simulink model "DAB_RA8P1_Final_Physical_MOSFET"  (R2024b)
settings: Solver=daessc  StartTime=0.0  StopTime=0.03  MaxStep=1e-8  RelTol=2e-3  AbsTol=1e-5
libraries: ee_lib x118, fl_lib x18, nesl_utility x15
(part 1 of 6)
Description:
  | H1.7 physical DAB model. Includes MOS/PCB/TMCS conductor parasitics, TMCS 120 ns + 1.1 MHz measurement path, 250 ns worst-case OC delay, hardware latch abstraction, independent driver enable, and physical-model EPS. TMCS1133B1A hardware mapping: 25 mV/A at 3.3 V; saved OC thresholds 63.728093 A primary and 39.169139 A secondary.
settings Model: Creator=LENOVO  LastModifiedBy=26488

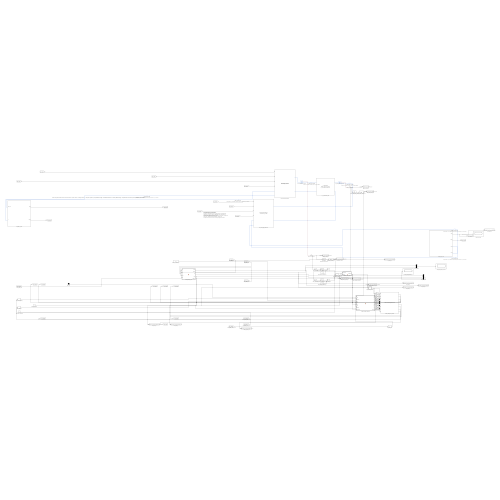
[thumbnail: Simulink's stored preview of the top-level diagram]
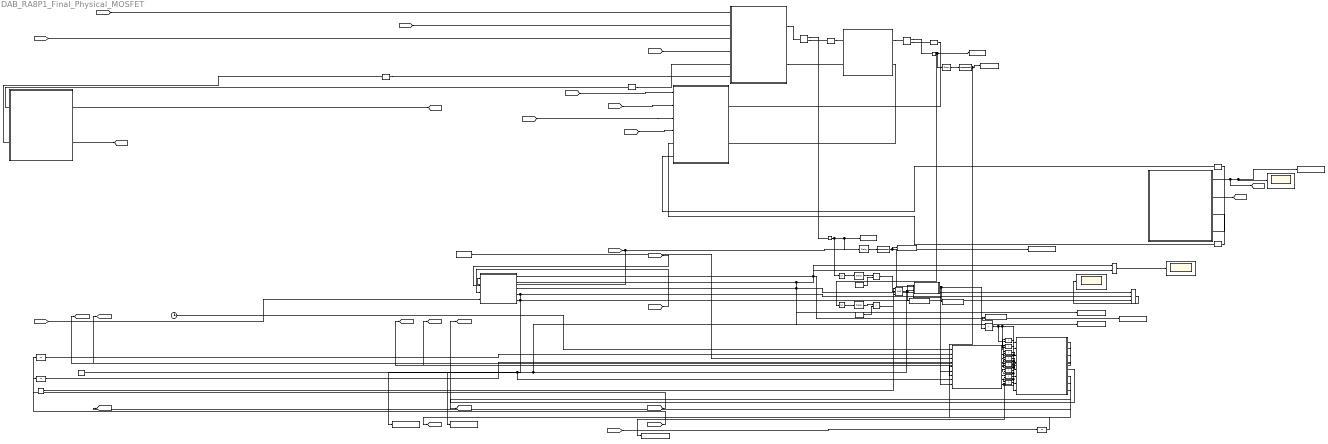
== system DAB_RA8P1_Final_Physical_MOSFET ==
  note: Selected physical parts used in the final model
      | Q1-Q8: AOS AONS66917, 100 V silicon MOSFET.
      | Gate drive: 4x UCC21520DWR, 0/10.18 V, 120 ns MCU dead time, no PNP/NPN booster.
      | Per MOS: Rg_on 4.7 Ohm, Rg_off 2.2 Ohm, PMEG4010ER, Rgs 10 kOhm, BZT52C15.
      | Transformer: custom PQ4040 PC95, Np:Ns=1:2 fixed, L1/L2=57.5/230uH, Llk_sec(total)=0.5uH.
      | Input CM choke only: 2mH per winding, 30A, no bypass.
      | Output: CSEC -> SER2915H-222KL 2.2uH/2.05mOhm -> 8000uF COUT.
      | No output common-mode choke, no common-mode copper bridge, no GaN variant.
  note: Power path: input EMI -> primary MOSFET full bridge -> PQ4040/PC95 transformer -> secondary MOSFET bridge -> output filter/load. Control and scopes are kept below the power schematic.
  note: RA8P1-friendly realtime feedback control: measured Vin/Vout/Iout -> PI phase command -> isolated gate interface.
  ADC_Delay_Iout : UnitDelay  SampleTime=1e-6  HasFrameUpgradeWarning=on
  ADC_Delay_Vin : UnitDelay  InitialCondition=24  SampleTime=1e-6  HasFrameUpgradeWarning=on
  ADC_OneCycle_Delay : UnitDelay  SampleTime=1e-6  HasFrameUpgradeWarning=on
  DRIVER_ENABLE_scope_sl : ToWorkspace  VariableName=DAB_RA8P1_Final_Physical_MOSFET_driver_enable  SaveFormat=Structure With Time  SampleTime=-1
  Eff_scope_sl : ToWorkspace  VariableName=DAB_RA8P1_Final_Physical_MOSFET_efficiency  SaveFormat=Structure With Time  SampleTime=-1
  FAULT_LATCH_N_scope_sl : ToWorkspace  VariableName=DAB_RA8P1_Final_Physical_MOSFET_fault_latch_n  SaveFormat=Structure With Time  SampleTime=-1
  HW_DRIVER_ENABLE : Product
  HW_GATE_Q{1..8} (8 alike) : Product
  Hardware_Fault_Latch_N : MATLAB Function  TreatAsAtomicUnit=on
  IPRI_Abs_For_OC : Abs  SaturateOnIntegerOverflow=off
  IPRI_HF_To_Simulink : nesl_utility/PS-Simulink Converter  PhysicalDomain=network_engine_domain  SubClassName=ps_output  LeftPortType=input  RightPortType=output  PseudoPeriodic=off  Frequencies=[]  VectorFormat=inherit  Unit=inherit  AffineConversion=off
  IPRI_HF_scope_sl : ToWorkspace  VariableName=DAB_RA8P1_Final_Physical_MOSFET_ipri_hf  SaveFormat=Structure With Time
  IPRI_HW_OC_Threshold_A : Constant  Value=63.728093
  IPRI_OC_Safe : RelationalOperator  Operator=<  OutDataTypeStr=boolean  RndMeth=Simplest  InputSameDT=off
  IPRI_TMCS_scope_sl : ToWorkspace  VariableName=DAB_RA8P1_Final_Physical_MOSFET_ipri_tmcs  SaveFormat=Structure With Time  SampleTime=-1
  ISEC_Abs_For_OC : Abs  SaturateOnIntegerOverflow=off
  ISEC_HF_To_Simulink : nesl_utility/PS-Simulink Converter  PhysicalDomain=network_engine_domain  SubClassName=ps_output  LeftPortType=input  RightPortType=output  PseudoPeriodic=off  Frequencies=[]  VectorFormat=inherit  Unit=inherit  AffineConversion=off
  ISEC_HF_scope_sl : ToWorkspace  VariableName=DAB_RA8P1_Final_Physical_MOSFET_isec_hf  SaveFormat=Structure With Time
  ISEC_HW_OC_Threshold_A : Constant  Value=39.169139
  ISEC_OC_Safe : RelationalOperator  Operator=<  OutDataTypeStr=boolean  RndMeth=Simplest  InputSameDT=off
  ISEC_TMCS_scope_sl : ToWorkspace  VariableName=DAB_RA8P1_Final_Physical_MOSFET_isec_tmcs  SaveFormat=Structure With Time  SampleTime=-1
  Iin_scope_sl : ToWorkspace  VariableName=DAB_RA8P1_Final_Physical_MOSFET_iin  SaveFormat=Structure With Time  SampleTime=-1
  Input_EMI_DC_Link : Subsystem
  Iout_scope_sl : ToWorkspace  VariableName=DAB_RA8P1_Final_Physical_MOSFET_iout  SaveFormat=Structure With Time  SampleTime=-1
  Isolated_Gate_Drive_Interface : Subsystem
      mask Display: color('black');disp('UCC21520 isolated gate driver bank');
  LPCB_PRI_NEG_5nH : ee_lib/Passive/Inductor  l=5 nH  enable_L_tol=ee.enum.toleranceApplication.none  L_tol=20  tol_distribution=ee.enum.toleranceDistribution.uniform  nSigma=4  r=0.0001 Ohm  g=1e-9 1/Ohm  enable_operating_limits=ee.enum.enable.no  operating_limit_action=ee.enum.passive.reportOpLim.warn  max_working_current=1 A  power_rating=1 W  fault_action=simscape.enum.assert.action.none  t_fault=1 s  i_L_specify=off  i_L_priority=High  i_L=0 A  i_L_nominal_specify=off  i_L_nominal_value=1  i_L_nominal_unit=A
      settings: AttributesFormatString=PCB parasitic only; not a BOM component; keep PRI local DC loop <=10nH total
  LPCB_PRI_POS_5nH : ee_lib/Passive/Inductor  l=5 nH  enable_L_tol=ee.enum.toleranceApplication.none  L_tol=20  tol_distribution=ee.enum.toleranceDistribution.uniform  nSigma=4  r=0.0001 Ohm  g=1e-9 1/Ohm  enable_operating_limits=ee.enum.enable.no  operating_limit_action=ee.enum.passive.reportOpLim.warn  max_working_current=1 A  power_rating=1 W  fault_action=simscape.enum.assert.action.none  t_fault=1 s  i_L_specify=off  i_L_priority=High  i_L=0 A  i_L_nominal_specify=off  i_L_nominal_value=1  i_L_nominal_unit=A
      settings: AttributesFormatString=PCB parasitic only; not a BOM component; keep PRI local DC loop <=10nH total
  LPCB_SEC_NEG_5nH : ee_lib/Passive/Inductor  l=5 nH  enable_L_tol=ee.enum.toleranceApplication.none  L_tol=20  tol_distribution=ee.enum.toleranceDistribution.uniform  nSigma=4  r=0.0001 Ohm  g=1e-9 1/Ohm  enable_operating_limits=ee.enum.enable.no  operating_limit_action=ee.enum.passive.reportOpLim.warn  max_working_current=1 A  power_rating=1 W  fault_action=simscape.enum.assert.action.none  t_fault=1 s  i_L_specify=off  i_L_priority=High  i_L=0 A  i_L_nominal_specify=off  i_L_nominal_value=1  i_L_nominal_unit=A
      settings: AttributesFormatString=PCB parasitic only; not a BOM component; keep SEC local DC loop <=10nH total
  LPCB_SEC_POS_5nH : ee_lib/Passive/Inductor  l=5 nH  enable_L_tol=ee.enum.toleranceApplication.none  L_tol=20  tol_distribution=ee.enum.toleranceDistribution.uniform  nSigma=4  r=0.0001 Ohm  g=1e-9 1/Ohm  enable_operating_limits=ee.enum.enable.no  operating_limit_action=ee.enum.passive.reportOpLim.warn  max_working_current=1 A  power_rating=1 W  fault_action=simscape.enum.assert.action.none  t_fault=1 s  i_L_specify=off  i_L_priority=High  i_L=0 A  i_L_nominal_specify=off  i_L_nominal_value=1  i_L_nominal_unit=A
      settings: AttributesFormatString=PCB parasitic only; not a BOM component; keep SEC local DC loop <=10nH total
  MCU_Vout_Setpoint_V : Constant  Value=48
  Mux_Currents : Mux  Inputs=2
  Mux_Power_Eff : Mux  Inputs=3
  Output_Filter_Load : Subsystem
  PRI_Full_Bridge_RealDrivers : Subsystem
      mask Display: color('black');disp('PRI Full Bridge RealDrivers\nnonideal FETs + gate RCD');
  Phase_us_scope_sl : ToWorkspace  VariableName=DAB_RA8P1_Final_Physical_MOSFET_phase_us  SaveFormat=Structure With Time  SampleTime=-1
  Pin_scope_sl : ToWorkspace  VariableName=DAB_RA8P1_Final_Physical_MOSFET_pin  SaveFormat=Structure With Time  SampleTime=-1
  Pout_scope_sl : ToWorkspace  VariableName=DAB_RA8P1_Final_Physical_MOSFET_pout  SaveFormat=Structure With Time  SampleTime=-1
  Power_Efficiency_Calc : MATLAB Function  TreatAsAtomicUnit=on
  RA8P1_Realtime_Voltage_PI : MATLAB Function  TreatAsAtomicUnit=on
  RAW_FAULT_N_Model : Constant
  RAW_FAULT_N_With_OC : Logic  Inputs=3  AllPortsSameDT=off  OutDataTypeStr=boolean
  RAW_FAULT_N_scope_sl : ToWorkspace  VariableName=DAB_RA8P1_Final_Physical_MOSFET_raw_fault_n  SaveFormat=Structure With Time  SampleTime=-1
  RUN_REQ_Model : Constant
  R_TMCS_PRI_0p7mOhm : ee_lib/Passive/Resistor  R=0.0007 Ohm  enable_R_tol=ee.enum.toleranceApplication.none  R_tol=5  tol_distribution=ee.enum.toleranceDistribution.uniform  nSigma=4  enable_operating_limits=ee.enum.enable.no  operating_limit_action=ee.enum.passive.reportOpLim.warn  power_rating=1 W  max_working_voltage=100 V  noise_mode=ee.enum.sources.noise.Disabled  Tdevice=25 degC  sample_time=1e-3 s  repeatability=ee.enum.ic.repeatability.notRepeatable  user_seed=0  auto_seed=3499211588  fault_action=simscape.enum.assert.action.none  t_fault=1 s  power_derating_T1=70 degC  power_derating_T2=155 degC  operating_temperature_range_vec=[-50, 150] degC  alpha=3.93e-3 1/K  Tmeas=25 degC  thermal_mass=100 J/K  temperature_specify=off  temperature_priority=High  temperature=298.15 K  temperature_nominal_specify=off  temperature_nominal_value=1  temperature_nominal_unit=K
      settings: AttributesFormatString=TMCS1133 conductor resistance; physical U_IPRI in BOM
  R_TMCS_SEC_0p7mOhm : ee_lib/Passive/Resistor  R=0.0007 Ohm  enable_R_tol=ee.enum.toleranceApplication.none  R_tol=5  tol_distribution=ee.enum.toleranceDistribution.uniform  nSigma=4  enable_operating_limits=ee.enum.enable.no  operating_limit_action=ee.enum.passive.reportOpLim.warn  power_rating=1 W  max_working_voltage=100 V  noise_mode=ee.enum.sources.noise.Disabled  Tdevice=25 degC  sample_time=1e-3 s  repeatability=ee.enum.ic.repeatability.notRepeatable  user_seed=0  auto_seed=3890346746  fault_action=simscape.enum.assert.action.none  t_fault=1 s  power_derating_T1=70 degC  power_derating_T2=155 degC  operating_temperature_range_vec=[-50, 150] degC  alpha=3.93e-3 1/K  Tmeas=25 degC  thermal_mass=100 J/K  temperature_specify=off  temperature_priority=High  temperature=298.15 K  temperature_nominal_specify=off  temperature_nominal_value=1  temperature_nominal_unit=K
      settings: AttributesFormatString=TMCS1133 conductor resistance; physical U_ISEC in BOM
  SEC_Full_Bridge_RealDrivers : Subsystem
      mask Display: color('black');disp('SEC Full Bridge RealDrivers\nnonideal FETs + gate RCD');
  Scope_Input_Output_Current : Scope
  Scope_Power_Efficiency : Scope
  Scope_Vout_Load : Scope
  Sim_Time : Clock
  T1_HF_Transformer_Real : Subsystem
      mask Display: color('black');disp('T1 PQ4040 PC95\nNp:Ns 1:2 fixed, Llk_sec 0.5uH\nLm_sec 230uH, DCR 0.95/3mR');
  TMCS_IPRI_1p1MHz_LPF : TransferFcn  Numerator=[2*pi*1.1e6]  Denominator=[1 2*pi*1.1e6]
  TMCS_IPRI_Analog_Delay : TransportDelay  DelayTime=120e-9
  TMCS_IPRI_OC_WorstCase_Delay : TransportDelay  DelayTime=250e-9
  TMCS_ISEC_1p1MHz_LPF : TransferFcn  Numerator=[2*pi*1.1e6]  Denominator=[1 2*pi*1.1e6]
  TMCS_ISEC_Analog_Delay : TransportDelay  DelayTime=120e-9
  TMCS_ISEC_OC_WorstCase_Delay : TransportDelay  DelayTime=250e-9
  U_IPRI_TMCS1133_Current : fl_lib/Electrical/Electrical Sensors/Current Sensor
  U_ISEC_TMCS1133_Current : fl_lib/Electrical/Electrical Sensors/Current Sensor
  Vin_scope_sl : ToWorkspace  VariableName=DAB_RA8P1_Final_Physical_MOSFET_vin  SaveFormat=Structure With Time  SampleTime=-1
  Vout_scope_sl : ToWorkspace  VariableName=DAB_RA8P1_Final_Physical_MOSFET_vout  SaveFormat=Structure With Time  SampleTime=-1
  wires:
  [VIN_MEAS] -> Power_Efficiency_Calc/1(Vin), Vin_scope_sl/1
  [IIN_MEAS] -> Power_Efficiency_Calc/2(Iin)
  [VOUT_MEAS] -> Power_Efficiency_Calc/3(Vout)
  [IOUT_MEAS] -> Power_Efficiency_Calc/4(Iout)
  Power_Efficiency_Calc/1(IinAbs) -> Iin_scope_sl/1, Mux_Currents/1
  Power_Efficiency_Calc/2(IoutAbs) -> Mux_Currents/2, Iout_scope_sl/1
  Power_Efficiency_Calc/3(Pin) -> Pin_scope_sl/1, Mux_Power_Eff/1
  Power_Efficiency_Calc/4(Pout) -> Pout_scope_sl/1, Mux_Power_Eff/2
  Power_Efficiency_Calc/5(Efficiency) -> Mux_Power_Eff/3, Eff_scope_sl/1
  Mux_Currents/1 -> Scope_Input_Output_Current/1
  Mux_Power_Eff/1 -> Scope_Power_Efficiency/1
  Input_EMI_DC_Link/1(output) -> [IIN_MEAS]
  Input_EMI_DC_Link/2(output1) -> [VIN_MEAS]
  Output_Filter_Load/1(output) -> Vout_scope_sl/1, Scope_Vout_Load/1, [VOUT_MEAS]
  Output_Filter_Load/2(output1) -> [IOUT_MEAS]
  Isolated_Gate_Drive_Interface/1(GATE_OUT_1) -> [Q1_GATE]
  Isolated_Gate_Drive_Interface/2(GATE_OUT_2) -> [Q2_GATE]
  Isolated_Gate_Drive_Interface/3(GATE_OUT_3) -> [Q3_GATE]
  Isolated_Gate_Drive_Interface/4(GATE_OUT_4) -> [Q4_GATE]
  Isolated_Gate_Drive_Interface/5(GATE_OUT_5) -> [Q5_GATE]
  Isolated_Gate_Drive_Interface/6(GATE_OUT_6) -> [Q6_GATE]
  Isolated_Gate_Drive_Interface/7(GATE_OUT_7) -> [Q7_GATE]
  Isolated_Gate_Drive_Interface/8(GATE_OUT_8) -> [Q8_GATE]
  Sim_Time/1 -> RA8P1_Realtime_Voltage_PI/1(t)
  ADC_OneCycle_Delay/1 -> RA8P1_Realtime_Voltage_PI/2(Vout)
  MCU_Vout_Setpoint_V/1 -> RA8P1_Realtime_Voltage_PI/3(VrefCmd)
  [VIN_MEAS] -> ADC_Delay_Vin/1
  ADC_Delay_Vin/1 -> RA8P1_Realtime_Voltage_PI/4(Vin)
  [IOUT_MEAS] -> ADC_Delay_Iout/1
  ADC_Delay_Iout/1 -> RA8P1_Realtime_Voltage_PI/5(Iout)
  RA8P1_Realtime_Voltage_PI/9(PhaseUs) -> Phase_us_scope_sl/1
  [Q1_GATE] -> PRI_Full_Bridge_RealDrivers/1(G1_A_HS)
  [Q2_GATE] -> PRI_Full_Bridge_RealDrivers/2(G2_A_LS)
  [Q3_GATE] -> PRI_Full_Bridge_RealDrivers/3(G3_B_HS)
  [Q4_GATE] -> PRI_Full_Bridge_RealDrivers/4(G4_B_LS)
  [Q5_GATE] -> SEC_Full_Bridge_RealDrivers/1(G1_A_HS)
  [Q6_GATE] -> SEC_Full_Bridge_RealDrivers/2(G2_A_LS)
  [Q7_GATE] -> SEC_Full_Bridge_RealDrivers/3(G3_B_HS)
  [Q8_GATE] -> SEC_Full_Bridge_RealDrivers/4(G4_B_LS)
  [VOUT_MEAS] -> ADC_OneCycle_Delay/1
  RUN_REQ_Model/1 -> Hardware_Fault_Latch_N/2(RunReq), HW_DRIVER_ENABLE/1, RA8P1_Realtime_Voltage_PI/8(RunReq)
  IPRI_HF_To_Simulink/1 -> IPRI_HF_scope_sl/1, TMCS_IPRI_Analog_Delay/1, IPRI_Abs_For_OC/1
  TMCS_IPRI_Analog_Delay/1 -> TMCS_IPRI_1p1MHz_LPF/1
  TMCS_IPRI_1p1MHz_LPF/1 -> RA8P1_Realtime_Voltage_PI/6(Ipri), IPRI_TMCS_scope_sl/1
  ISEC_HF_To_Simulink/1 -> ISEC_HF_scope_sl/1, TMCS_ISEC_Analog_Delay/1, ISEC_Abs_For_OC/1
  TMCS_ISEC_Analog_Delay/1 -> TMCS_ISEC_1p1MHz_LPF/1
  TMCS_ISEC_1p1MHz_LPF/1 -> RA8P1_Realtime_Voltage_PI/7(Isec), ISEC_TMCS_scope_sl/1
  IPRI_Abs_For_OC/1 -> TMCS_IPRI_OC_WorstCase_Delay/1
  TMCS_IPRI_OC_WorstCase_Delay/1 -> IPRI_OC_Safe/1
  IPRI_HW_OC_Threshold_A/1 -> IPRI_OC_Safe/2
  ISEC_Abs_For_OC/1 -> TMCS_ISEC_OC_WorstCase_Delay/1
  TMCS_ISEC_OC_WorstCase_Delay/1 -> ISEC_OC_Safe/1
  ISEC_HW_OC_Threshold_A/1 -> ISEC_OC_Safe/2
  RAW_FAULT_N_Model/1 -> RAW_FAULT_N_With_OC/1
  IPRI_OC_Safe/1 -> RAW_FAULT_N_With_OC/2
  ISEC_OC_Safe/1 -> RAW_FAULT_N_With_OC/3
  RAW_FAULT_N_With_OC/1 -> RAW_FAULT_N_scope_sl/1, Hardware_Fault_Latch_N/1(RawFaultN)
  Hardware_Fault_Latch_N/1(FaultLatchN) -> FAULT_LATCH_N_scope_sl/1, HW_DRIVER_ENABLE/2, RA8P1_Realtime_Voltage_PI/9(RawFaultN)
  HW_DRIVER_ENABLE/1 -> HW_GATE_Q7/2, HW_GATE_Q8/2, HW_GATE_Q6/2, HW_GATE_Q5/2, HW_GATE_Q4/2, HW_GATE_Q3/2, HW_GATE_Q2/2, HW_GATE_Q1/2, DRIVER_ENABLE_scope_sl/1
  RA8P1_Realtime_Voltage_PI/1(g1) -> HW_GATE_Q1/1
  HW_GATE_Q1/1 -> Isolated_Gate_Drive_Interface/1(PWM_IN_1)
  RA8P1_Realtime_Voltage_PI/2(g2) -> HW_GATE_Q2/1
  HW_GATE_Q2/1 -> Isolated_Gate_Drive_Interface/2(PWM_IN_2)
  RA8P1_Realtime_Voltage_PI/3(g3) -> HW_GATE_Q3/1
  HW_GATE_Q3/1 -> Isolated_Gate_Drive_Interface/3(PWM_IN_3)
  RA8P1_Realtime_Voltage_PI/4(g4) -> HW_GATE_Q4/1
  HW_GATE_Q4/1 -> Isolated_Gate_Drive_Interface/4(PWM_IN_4)
  RA8P1_Realtime_Voltage_PI/5(g5) -> HW_GATE_Q5/1
  HW_GATE_Q5/1 -> Isolated_Gate_Drive_Interface/5(PWM_IN_5)
  RA8P1_Realtime_Voltage_PI/6(g6) -> HW_GATE_Q6/1
  HW_GATE_Q6/1 -> Isolated_Gate_Drive_Interface/6(PWM_IN_6)
  RA8P1_Realtime_Voltage_PI/7(g7) -> HW_GATE_Q7/1
  HW_GATE_Q7/1 -> Isolated_Gate_Drive_Interface/7(PWM_IN_7)
  RA8P1_Realtime_Voltage_PI/8(g8) -> HW_GATE_Q8/1
  HW_GATE_Q8/1 -> Isolated_Gate_Drive_Interface/8(PWM_IN_8)
  connections:
  PRI_Full_Bridge_RealDrivers/RConn2 -- T1_HF_Transformer_Real/LConn2
  T1_HF_Transformer_Real/RConn2 -- SEC_Full_Bridge_RealDrivers/RConn2
  Input_EMI_DC_Link/LConn1 -- LPCB_PRI_POS_5nH/LConn1
  LPCB_PRI_POS_5nH/RConn1 -- PRI_Full_Bridge_RealDrivers/LConn1
  Input_EMI_DC_Link/LConn2 -- LPCB_PRI_NEG_5nH/LConn1
  LPCB_PRI_NEG_5nH/RConn1 -- PRI_Full_Bridge_RealDrivers/LConn2
  SEC_Full_Bridge_RealDrivers/LConn1 -- LPCB_SEC_POS_5nH/LConn1
  LPCB_SEC_POS_5nH/RConn1 -- Output_Filter_Load/RConn1
  SEC_Full_Bridge_RealDrivers/LConn2 -- LPCB_SEC_NEG_5nH/LConn1
  LPCB_SEC_NEG_5nH/RConn1 -- Output_Filter_Load/RConn2
  PRI_Full_Bridge_RealDrivers/RConn1 -- U_IPRI_TMCS1133_Current/LConn1
  U_IPRI_TMCS1133_Current/RConn2 -- R_TMCS_PRI_0p7mOhm/LConn1
  R_TMCS_PRI_0p7mOhm/RConn1 -- T1_HF_Transformer_Real/LConn1
  T1_HF_Transformer_Real/RConn1 -- U_ISEC_TMCS1133_Current/LConn1
  U_ISEC_TMCS1133_Current/RConn2 -- R_TMCS_SEC_0p7mOhm/LConn1
  R_TMCS_SEC_0p7mOhm/RConn1 -- SEC_Full_Bridge_RealDrivers/RConn1
  U_IPRI_TMCS1133_Current/RConn1 -- IPRI_HF_To_Simulink/LConn1
  U_ISEC_TMCS1133_Current/RConn1 -- ISEC_HF_To_Simulink/LConn1

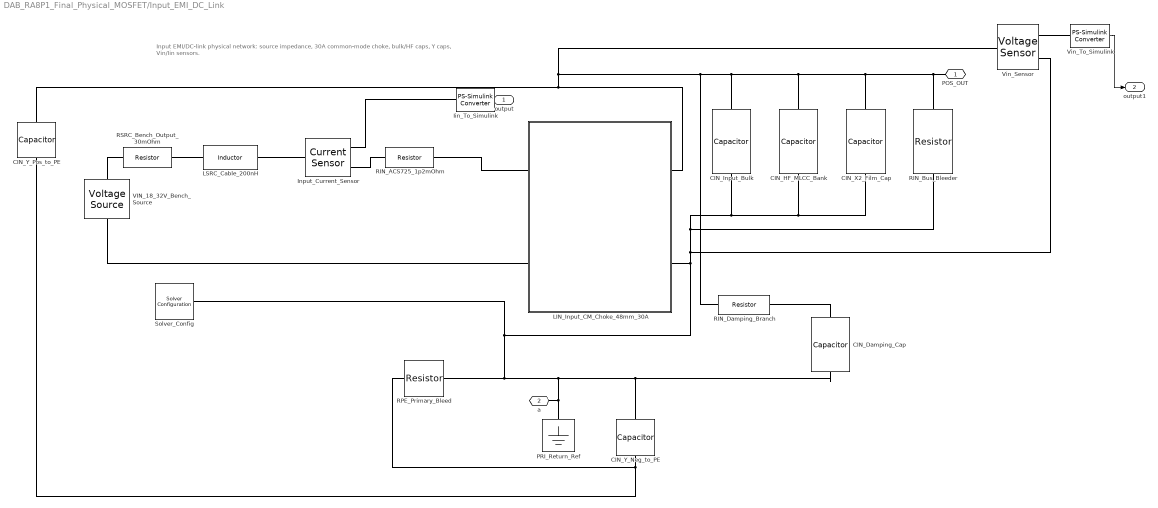
== system DAB_RA8P1_Final_Physical_MOSFET/Input_EMI_DC_Link ==
  note: Input EMI/DC-link physical network: source impedance, 30A common-mode choke, bulk/HF caps, Y caps, Vin/Iin sensors.
  CIN_Damping_Cap : ee_lib/Passive/Capacitor  cap_option=ee.enum.passive.capacitor.capOption.const  c=40 uF  Cvec=[1e-05, 1e-06] F  Vvec=[0, 10] V  CV_table_symmetry=ee.enum.passive.capacitor.tableSymmetry.yes  f_vec=[1, 10] kHz  DFext_vec=[.8, 1.2]  enable_C_tol=ee.enum.toleranceApplication.none  averaging_period=0 s  C_tol=5  tol_distribution=ee.enum.toleranceDistribution.uniform  nSigma=4  r=0.002 Ohm  g=0 1/Ohm  enable_operating_limits=ee.enum.enable.no  operating_limit_action=ee.enum.passive.reportOpLim.warn  max_working_voltage_range=[-25, 25] V  power_rating=1 W  maxTemperature=85 degC  thermalEnable=false  thermalMass=1 J/K  fault_action=simscape.enum.assert.action.none  t_fault=1 s  i_specify=off  i_priority=None  i=0 A  i_nominal_specify=off  i_nominal_value=1  i_nominal_unit=A  v_specify=off  v_priority=None  v=0 V  v_nominal_specify=off  v_nominal_value=1  v_nominal_unit=V  vc_specify=on  vc_priority=High  vc=24 V  vc_nominal_specify=off  vc_nominal_value=1  vc_nominal_unit=V  T_specify=off  T_priority=None  T=298.15 K  T_nominal_specify=off  T_nominal_value=1  T_nominal_unit=K
      settings: AttributesFormatString=110uF
  CIN_HF_MLCC_Bank : ee_lib/Passive/Capacitor  cap_option=ee.enum.passive.capacitor.capOption.const  c=220 uF  Cvec=[1e-05, 1e-06] F  Vvec=[0, 10] V  CV_table_symmetry=ee.enum.passive.capacitor.tableSymmetry.yes  f_vec=[1, 10] kHz  DFext_vec=[.8, 1.2]  enable_C_tol=ee.enum.toleranceApplication.none  averaging_period=0 s  C_tol=5  tol_distribution=ee.enum.toleranceDistribution.uniform  nSigma=4  r=0.0010 Ohm  g=0 1/Ohm  enable_operating_limits=ee.enum.enable.no  operating_limit_action=ee.enum.passive.reportOpLim.warn  max_working_voltage_range=[-25, 25] V  power_rating=1 W  maxTemperature=85 degC  thermalEnable=false  thermalMass=1 J/K  fault_action=simscape.enum.assert.action.none  t_fault=1 s  i_specify=off  i_priority=None  i=0 A  i_nominal_specify=off  i_nominal_value=1  i_nominal_unit=A  v_specify=off  v_priority=None  v=0 V  v_nominal_specify=off  v_nominal_value=1  v_nominal_unit=V  vc_specify=on  vc_priority=High  vc=24 V  vc_nominal_specify=off  vc_nominal_value=1  vc_nominal_unit=V  T_specify=off  T_priority=None  T=298.15 K  T_nominal_specify=off  T_nominal_value=1  T_nominal_unit=K
      settings: AttributesFormatString=220uF\nMLCC
  CIN_Input_Bulk : ee_lib/Passive/Capacitor  cap_option=ee.enum.passive.capacitor.capOption.const  c=4000 uF  Cvec=[1e-05, 1e-06] F  Vvec=[0, 10] V  CV_table_symmetry=ee.enum.passive.capacitor.tableSymmetry.yes  f_vec=[1, 10] kHz  DFext_vec=[.8, 1.2]  enable_C_tol=ee.enum.toleranceApplication.none  averaging_period=0 s  C_tol=5  tol_distribution=ee.enum.toleranceDistribution.uniform  nSigma=4  r=0.006 Ohm  g=0 1/Ohm  enable_operating_limits=ee.enum.enable.no  operating_limit_action=ee.enum.passive.reportOpLim.warn  max_working_voltage_range=[-25, 25] V  power_rating=1 W  maxTemperature=85 degC  thermalEnable=false  thermalMass=1 J/K  fault_action=simscape.enum.assert.action.none  t_fault=1 s  i_specify=off  i_priority=None  i=0 A  i_nominal_specify=off  i_nominal_value=1  i_nominal_unit=A  v_specify=off  v_priority=None  v=0 V  v_nominal_specify=off  v_nominal_value=1  v_nominal_unit=V  vc_specify=on  vc_priority=High  vc=24 V  vc_nominal_specify=off  vc_nominal_value=1  vc_nominal_unit=V  T_specify=off  T_priority=None  T=298.15 K  T_nominal_specify=off  T_nominal_value=1  T_nominal_unit=K
      settings: AttributesFormatString=4000uF\nESR 6mR
  CIN_X2_Film_Cap : ee_lib/Passive/Capacitor  cap_option=ee.enum.passive.capacitor.capOption.const  c=2.2 uF  Cvec=[1e-05, 1e-06] F  Vvec=[0, 10] V  CV_table_symmetry=ee.enum.passive.capacitor.tableSymmetry.yes  f_vec=[1, 10] kHz  DFext_vec=[.8, 1.2]  enable_C_tol=ee.enum.toleranceApplication.none  averaging_period=0 s  C_tol=5  tol_distribution=ee.enum.toleranceDistribution.uniform  nSigma=4  r=0.01 Ohm  g=0 1/Ohm  enable_operating_limits=ee.enum.enable.no  operating_limit_action=ee.enum.passive.reportOpLim.warn  max_working_voltage_range=[-25, 25] V  power_rating=1 W  maxTemperature=85 degC  thermalEnable=false  thermalMass=1 J/K  fault_action=simscape.enum.assert.action.none  t_fault=1 s  i_specify=off  i_priority=None  i=0 A  i_nominal_specify=off  i_nominal_value=1  i_nominal_unit=A  v_specify=off  v_priority=None  v=0 V  v_nominal_specify=off  v_nominal_value=1  v_nominal_unit=V  vc_specify=on  vc_priority=High  vc=24 V  vc_nominal_specify=off  vc_nominal_value=1  vc_nominal_unit=V  T_specify=off  T_priority=None  T=298.15 K  T_nominal_specify=off  T_nominal_value=1  T_nominal_unit=K
      settings: AttributesFormatString=2.2uF film
  CIN_Y_Neg_to_PE : ee_lib/Passive/Capacitor  cap_option=ee.enum.passive.capacitor.capOption.const  c=2.2 nF  Cvec=[1e-05, 1e-06] F  Vvec=[0, 10] V  CV_table_symmetry=ee.enum.passive.capacitor.tableSymmetry.yes  f_vec=[1, 10] kHz  DFext_vec=[.8, 1.2]  enable_C_tol=ee.enum.toleranceApplication.none  averaging_period=0 s  C_tol=5  tol_distribution=ee.enum.toleranceDistribution.uniform  nSigma=4  r=0.02 Ohm  g=0 1/Ohm  enable_operating_limits=ee.enum.enable.no  operating_limit_action=ee.enum.passive.reportOpLim.warn  max_working_voltage_range=[-25, 25] V  power_rating=1 W  maxTemperature=85 degC  thermalEnable=false  thermalMass=1 J/K  fault_action=simscape.enum.assert.action.none  t_fault=1 s  i_specify=off  i_priority=None  i=0 A  i_nominal_specify=off  i_nominal_value=1  i_nominal_unit=A  v_specify=off  v_priority=None  v=0 V  v_nominal_specify=off  v_nominal_value=1  v_nominal_unit=V  vc_specify=off  vc_priority=High  vc=0 V  vc_nominal_specify=off  vc_nominal_value=1  vc_nominal_unit=V  T_specify=off  T_priority=None  T=298.15 K  T_nominal_specify=off  T_nominal_value=1  T_nominal_unit=K
      settings: AttributesFormatString=Y 2.2nF
  CIN_Y_Pos_to_PE : ee_lib/Passive/Capacitor  cap_option=ee.enum.passive.capacitor.capOption.const  c=2.2 nF  Cvec=[1e-05, 1e-06] F  Vvec=[0, 10] V  CV_table_symmetry=ee.enum.passive.capacitor.tableSymmetry.yes  f_vec=[1, 10] kHz  DFext_vec=[.8, 1.2]  enable_C_tol=ee.enum.toleranceApplication.none  averaging_period=0 s  C_tol=5  tol_distribution=ee.enum.toleranceDistribution.uniform  nSigma=4  r=0.02 Ohm  g=0 1/Ohm  enable_operating_limits=ee.enum.enable.no  operating_limit_action=ee.enum.passive.reportOpLim.warn  max_working_voltage_range=[-25, 25] V  power_rating=1 W  maxTemperature=85 degC  thermalEnable=false  thermalMass=1 J/K  fault_action=simscape.enum.assert.action.none  t_fault=1 s  i_specify=off  i_priority=None  i=0 A  i_nominal_specify=off  i_nominal_value=1  i_nominal_unit=A  v_specify=off  v_priority=None  v=0 V  v_nominal_specify=off  v_nominal_value=1  v_nominal_unit=V  vc_specify=off  vc_priority=High  vc=0 V  vc_nominal_specify=off  vc_nominal_value=1  vc_nominal_unit=V  T_specify=off  T_priority=None  T=298.15 K  T_nominal_specify=off  T_nominal_value=1  T_nominal_unit=K
      settings: AttributesFormatString=Y 2.2nF
  Iin_To_Simulink : nesl_utility/PS-Simulink Converter  PhysicalDomain=network_engine_domain  SubClassName=ps_output  LeftPortType=input  RightPortType=output  PseudoPeriodic=off  Frequencies=[]  VectorFormat=inherit  Unit=inherit  AffineConversion=off
  Input_Current_Sensor : fl_lib/Electrical/Electrical Sensors/Current Sensor
      settings: AttributesFormatString=Iin sense
  LIN_Input_CM_Choke_48mm_30A : Subsystem
      mask Display: color('black');disp('48mm CM choke\n2mH, 30A, DCR<=3.5mR\nZcm>2.1k@150kHz');
  LSRC_Cable_200nH : ee_lib/Passive/Inductor  l=0.2 uH  enable_L_tol=ee.enum.toleranceApplication.none  L_tol=20  tol_distribution=ee.enum.toleranceDistribution.uniform  nSigma=4  r=0.003 Ohm  g=1e-9 1/Ohm  enable_operating_limits=ee.enum.enable.no  operating_limit_action=ee.enum.passive.reportOpLim.warn  max_working_current=50 A  power_rating=1 W  fault_action=simscape.enum.assert.action.none  t_fault=1 s  i_L_specify=off  i_L_priority=High  i_L=0 A  i_L_nominal_specify=off  i_L_nominal_value=1  i_L_nominal_unit=A
      settings: AttributesFormatString=200nH\n3mR
  PRI_Return_Ref : fl_lib/Electrical/Electrical Elements/Electrical Reference
  RIN_ACS725_1p2mOhm : ee_lib/Passive/Resistor  R=0.0012 Ohm  enable_R_tol=ee.enum.toleranceApplication.none  R_tol=5  tol_distribution=ee.enum.toleranceDistribution.uniform  nSigma=4  enable_operating_limits=ee.enum.enable.no  operating_limit_action=ee.enum.passive.reportOpLim.warn  power_rating=1 W  max_working_voltage=100 V  noise_mode=ee.enum.sources.noise.Disabled  Tdevice=25 degC  sample_time=1e-3 s  repeatability=ee.enum.ic.repeatability.notRepeatable  user_seed=0  auto_seed=3936355183  fault_action=simscape.enum.assert.action.none  t_fault=1 s  power_derating_T1=70 degC  power_derating_T2=155 degC  operating_temperature_range_vec=[-50, 150] degC  alpha=3.93e-3 1/K  Tmeas=25 degC  thermal_mass=100 J/K  temperature_specify=off  temperature_priority=High  temperature=298.15 K  temperature_nominal_specify=off  temperature_nominal_value=1  temperature_nominal_unit=K
      settings: AttributesFormatString=1mR
  RIN_Bus_Bleeder : ee_lib/Passive/Resistor  R=5000 Ohm  enable_R_tol=ee.enum.toleranceApplication.none  R_tol=5  tol_distribution=ee.enum.toleranceDistribution.uniform  nSigma=4  enable_operating_limits=ee.enum.enable.no  operating_limit_action=ee.enum.passive.reportOpLim.warn  power_rating=1 W  max_working_voltage=100 V  noise_mode=ee.enum.sources.noise.Disabled  Tdevice=25 degC  sample_time=1e-3 s  repeatability=ee.enum.ic.repeatability.notRepeatable  user_seed=0  auto_seed=1207334858  fault_action=simscape.enum.assert.action.none  t_fault=1 s  power_derating_T1=70 degC  power_derating_T2=155 degC  operating_temperature_range_vec=[-50, 150] degC  alpha=3.93e-3 1/K  Tmeas=25 degC  thermal_mass=100 J/K  temperature_specify=off  temperature_priority=High  temperature=298.15 K  temperature_nominal_specify=off  temperature_nominal_value=1  temperature_nominal_unit=K
      settings: AttributesFormatString=100k
  RIN_Damping_Branch : ee_lib/Passive/Resistor  R=0.33 Ohm  enable_R_tol=ee.enum.toleranceApplication.none  R_tol=5  tol_distribution=ee.enum.toleranceDistribution.uniform  nSigma=4  enable_operating_limits=ee.enum.enable.no  operating_limit_action=ee.enum.passive.reportOpLim.warn  power_rating=1 W  max_working_voltage=100 V  noise_mode=ee.enum.sources.noise.Disabled  Tdevice=25 degC  sample_time=1e-3 s  repeatability=ee.enum.ic.repeatability.notRepeatable  user_seed=0  auto_seed=3897705473  fault_action=simscape.enum.assert.action.none  t_fault=1 s  power_derating_T1=70 degC  power_derating_T2=155 degC  operating_temperature_range_vec=[-50, 150] degC  alpha=3.93e-3 1/K  Tmeas=25 degC  thermal_mass=100 J/K  temperature_specify=off  temperature_priority=High  temperature=298.15 K  temperature_nominal_specify=off  temperature_nominal_value=1  temperature_nominal_unit=K
      settings: AttributesFormatString=0.33R
  RPE_Primary_Bleed : ee_lib/Passive/Resistor  R=100000000 Ohm  enable_R_tol=ee.enum.toleranceApplication.none  R_tol=5  tol_distribution=ee.enum.toleranceDistribution.uniform  nSigma=4  enable_operating_limits=ee.enum.enable.no  operating_limit_action=ee.enum.passive.reportOpLim.warn  power_rating=1 W  max_working_voltage=100 V  noise_mode=ee.enum.sources.noise.Disabled  Tdevice=25 degC  sample_time=1e-3 s  repeatability=ee.enum.ic.repeatability.notRepeatable  user_seed=0  auto_seed=477115713  fault_action=simscape.enum.assert.action.none  t_fault=1 s  power_derating_T1=70 degC  power_derating_T2=155 degC  operating_temperature_range_vec=[-50, 150] degC  alpha=3.93e-3 1/K  Tmeas=25 degC  thermal_mass=100 J/K  temperature_specify=off  temperature_priority=High  temperature=298.15 K  temperature_nominal_specify=off  temperature_nominal_value=1  temperature_nominal_unit=K
      settings: AttributesFormatString=100MR
  RSRC_Bench_Output_30mOhm : ee_lib/Passive/Resistor  R=0.03 Ohm  enable_R_tol=ee.enum.toleranceApplication.none  R_tol=5  tol_distribution=ee.enum.toleranceDistribution.uniform  nSigma=4  enable_operating_limits=ee.enum.enable.no  operating_limit_action=ee.enum.passive.reportOpLim.warn  power_rating=1 W  max_working_voltage=100 V  noise_mode=ee.enum.sources.noise.Disabled  Tdevice=25 degC  sample_time=1e-3 s  repeatability=ee.enum.ic.repeatability.notRepeatable  user_seed=0  auto_seed=1331131015  fault_action=simscape.enum.assert.action.none  t_fault=1 s  power_derating_T1=70 degC  power_derating_T2=155 degC  operating_temperature_range_vec=[-50, 150] degC  alpha=3.93e-3 1/K  Tmeas=25 degC  thermal_mass=100 J/K  temperature_specify=off  temperature_priority=High  temperature=298.15 K  temperature_nominal_specify=off  temperature_nominal_value=1  temperature_nominal_unit=K
      settings: AttributesFormatString=30mR
  Solver_Config : nesl_utility/Solver Configuration  PhysicalDomain=network_engine_domain  SubClassName=solver  LeftPortType=input  RightPortType=generic  Tones=[]  Harmonics=[]  SimulateNoise=off  Profile=off  UseLocalSampling=off  EnableSwitchedLinearOptims=on  FrequencyDomain=off  UseCCode=off  RelTol=0.001  AbsTol=0.001  MinStep=1e-09  ToWorkspace=off  RevertToSquareIcSolve=off  NumHomotopyIterations=100  PhasorMode=off  PhasorModeNumHarmonics=1  ConsistencySolver=NEWTON_XTOL_AFTER_FTOL  IndexReductionMethod=DerivativeReplacement  DoDC=off  ResidualTolerance=1e-09  ConsistencyTolSource=LOCAL  ConsistencyAbsTol=1e-4  ConsistencyRelTol=1e-4  ConsistencyTolFactor=0.001  UseLocalSolver=on  LocalSolverChoice=NE_BACKWARD_EULER_ADVANCER  ResolveIndetEquations=on  FunctionEvalNumThread=1  LocalSolverSampleTime=5e-8  DoFixedCost=off  MaxNonlinIter=2  MaxModeIter=2  ComputeImpulses=off  ImpulseIterations=2  LinearAlgebra=auto  LinearAlgebraNumThread=0  EquationFormulation=NE_TIME_EF  DelaysMemoryBudget=1024  AutomaticFiltering=on  FilteringTimeConstant=0.001  PartitionStorageMethod=AS_NEEDED  PartitionMemoryBudget=1024  PartitionMethod=ROBUST  MultibodyUseLocalSolver=off  MultibodyLocalSolverChoice=ODE1  MultibodyLocalSolverSampleTime=0.001
  VIN_18_32V_Bench_Source : ee_lib/Sources/Voltage Source  dc_voltage=24 V  ac_voltage=0 V  ac_shift=0 rad  ac_frequency=60 Hz  noise_mode=ee.enum.sources.noise.Disabled  PSD=0 V^2/Hz  sample_time=1e-3 s  repeatability=ee.enum.sources.repeatability.NotRepeatable  user_seed=0  auto_seed=3208416576  i_specify=off  i_priority=None  i=0 A  i_nominal_specify=off  i_nominal_value=1  i_nominal_unit=A  v_specify=off  v_priority=None  v=0 V  v_nominal_specify=off  v_nominal_value=1  v_nominal_unit=V
      settings: AttributesFormatString=Vin 18-32V
  Vin_Sensor : fl_lib/Electrical/Electrical Sensors/Voltage Sensor
      settings: AttributesFormatString=Vin sense
  Vin_To_Simulink : nesl_utility/PS-Simulink Converter  PhysicalDomain=network_engine_domain  SubClassName=ps_output  LeftPortType=input  RightPortType=output  PseudoPeriodic=off  Frequencies=[]  VectorFormat=inherit  Unit=inherit  AffineConversion=off
  POS_OUT : PMIOPort  Side=Left
  a : PMIOPort  Port=2  Side=Left
  output : Outport
  output1 : Outport  Port=2
  wires:
  Iin_To_Simulink/1 -> output/1
  Vin_To_Simulink/1 -> output1/1
  connections:
  LIN_Input_CM_Choke_48mm_30A/RConn1 -- Vin_Sensor/LConn1 -- POS_OUT/RConn1 -- RIN_Bus_Bleeder/LConn1 -- CIN_X2_Film_Cap/LConn1 -- CIN_HF_MLCC_Bank/LConn1 -- CIN_Input_Bulk/LConn1 -- RIN_Damping_Branch/LConn1 -- CIN_Y_Pos_to_PE/LConn1
  CIN_Y_Pos_to_PE/RConn1 -- CIN_Y_Neg_to_PE/RConn1 -- RPE_Primary_Bleed/LConn1
  Input_Current_Sensor/RConn1 -- Iin_To_Simulink/LConn1
  VIN_18_32V_Bench_Source/LConn1 -- RSRC_Bench_Output_30mOhm/LConn1
  RPE_Primary_Bleed/RConn1 -- PRI_Return_Ref/LConn1 -- a/RConn1 -- CIN_Damping_Cap/RConn1 -- CIN_Y_Neg_to_PE/LConn1 -- Solver_Config/RConn1 -- Vin_Sensor/RConn2 -- CIN_X2_Film_Cap/RConn1 -- CIN_HF_MLCC_Bank/RConn1 -- CIN_Input_Bulk/RConn1 -- RIN_Bus_Bleeder/RConn1 -- LIN_Input_CM_Choke_48mm_30A/RConn2
  Vin_Sensor/RConn1 -- Vin_To_Simulink/LConn1
  RIN_Damping_Branch/RConn1 -- CIN_Damping_Cap/LConn1
  VIN_18_32V_Bench_Source/RConn1 -- LIN_Input_CM_Choke_48mm_30A/LConn2
  LSRC_Cable_200nH/RConn1 -- Input_Current_Sensor/LConn1
  Input_Current_Sensor/RConn2 -- RIN_ACS725_1p2mOhm/LConn1
  RIN_ACS725_1p2mOhm/RConn1 -- LIN_Input_CM_Choke_48mm_30A/LConn1
  RSRC_Bench_Output_30mOhm/RConn1 -- LSRC_Cable_200nH/LConn1

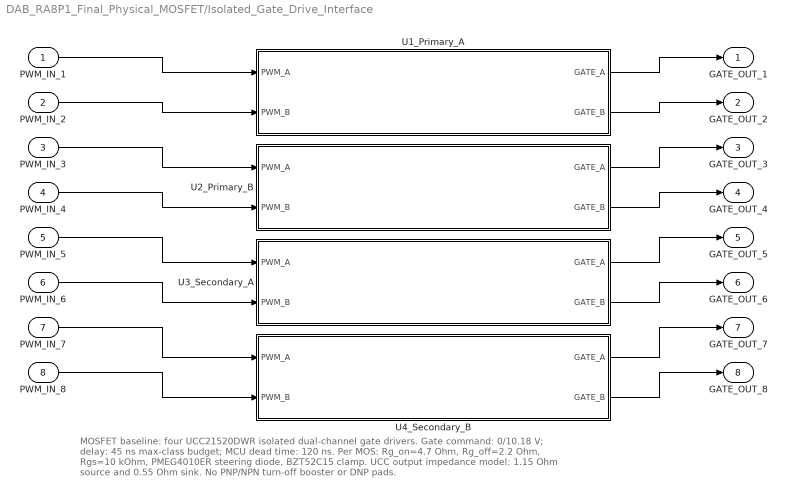
== system DAB_RA8P1_Final_Physical_MOSFET/Isolated_Gate_Drive_Interface ==
  note: MOSFET baseline: four UCC21520DWR isolated dual-channel gate drivers.
      | Gate command: 0/10.18 V; delay: 45 ns max-class budget; MCU dead time: 120 ns.
      | Per MOS: Rg_on=4.7 Ohm, Rg_off=2.2 Ohm, Rgs=10 kOhm, PMEG4010ER steering diode, BZT52C15 clamp.
      | UCC output impedance model: 1.15 Ohm source and 0.55 Ohm sink. No PNP/NPN turn-off booster or DNP pads.
  PWM_IN_1 : Inport
  PWM_IN_2 : Inport  Port=2
  PWM_IN_3 : Inport  Port=3
  PWM_IN_4 : Inport  Port=4
  PWM_IN_5 : Inport  Port=5
  PWM_IN_6 : Inport  Port=6
  PWM_IN_7 : Inport  Port=7
  PWM_IN_8 : Inport  Port=8
  U1_Primary_A : Subsystem
      mask Display: color('black');disp('UCC21520 dual isolated gate driver');
  U2_Primary_B : Subsystem
      mask Display: color('black');disp('UCC21520 dual isolated gate driver');
  U3_Secondary_A : Subsystem
      mask Display: color('black');disp('UCC21520 dual isolated gate driver');
  U4_Secondary_B : Subsystem
      mask Display: color('black');disp('UCC21520 dual isolated gate driver');
  GATE_OUT_1 : Outport
  GATE_OUT_2 : Outport  Port=2
  GATE_OUT_3 : Outport  Port=3
  GATE_OUT_4 : Outport  Port=4
  GATE_OUT_5 : Outport  Port=5
  GATE_OUT_6 : Outport  Port=6
  GATE_OUT_7 : Outport  Port=7
  GATE_OUT_8 : Outport  Port=8
  wires:
  PWM_IN_1/1 -> U1_Primary_A/1(PWM_A)
  PWM_IN_2/1 -> U1_Primary_A/2(PWM_B)
  U1_Primary_A/1(GATE_A) -> GATE_OUT_1/1
  U1_Primary_A/2(GATE_B) -> GATE_OUT_2/1
  PWM_IN_3/1 -> U2_Primary_B/1(PWM_A)
  PWM_IN_4/1 -> U2_Primary_B/2(PWM_B)
  U2_Primary_B/1(GATE_A) -> GATE_OUT_3/1
  U2_Primary_B/2(GATE_B) -> GATE_OUT_4/1
  PWM_IN_5/1 -> U3_Secondary_A/1(PWM_A)
  PWM_IN_6/1 -> U3_Secondary_A/2(PWM_B)
  U3_Secondary_A/1(GATE_A) -> GATE_OUT_5/1
  U3_Secondary_A/2(GATE_B) -> GATE_OUT_6/1
  PWM_IN_7/1 -> U4_Secondary_B/1(PWM_A)
  PWM_IN_8/1 -> U4_Secondary_B/2(PWM_B)
  U4_Secondary_B/1(GATE_A) -> GATE_OUT_7/1
  U4_Secondary_B/2(GATE_B) -> GATE_OUT_8/1

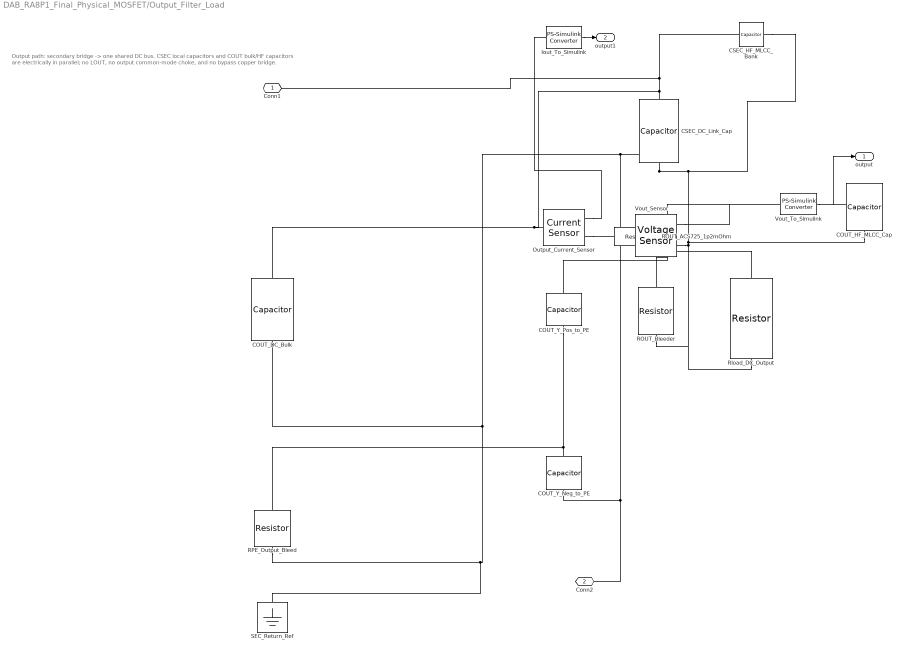
== system DAB_RA8P1_Final_Physical_MOSFET/Output_Filter_Load ==
  note: Output path: secondary bridge -> one shared DC bus. CSEC local capacitors and COUT bulk/HF capacitors are electrically in parallel; no LOUT, no output common-mode choke, and no bypass copper bridge.
  COUT_DC_Bulk : ee_lib/Passive/Capacitor  cap_option=ee.enum.passive.capacitor.capOption.const  c=4000 uF  Cvec=[1e-05, 1e-06] F  Vvec=[0, 10] V  CV_table_symmetry=ee.enum.passive.capacitor.tableSymmetry.yes  f_vec=[1, 10] kHz  DFext_vec=[.8, 1.2]  enable_C_tol=ee.enum.toleranceApplication.none  averaging_period=0 s  C_tol=5  tol_distribution=ee.enum.toleranceDistribution.uniform  nSigma=4  r=0.00775 Ohm  g=0 1/Ohm  enable_operating_limits=ee.enum.enable.no  operating_limit_action=ee.enum.passive.reportOpLim.warn  max_working_voltage_range=[-100,100] V  power_rating=1 W  maxTemperature=85 degC  thermalEnable=false  thermalMass=1 J/K  fault_action=simscape.enum.assert.action.none  t_fault=1 s  i_specify=off  i_priority=None  i=0 A  i_nominal_specify=off  i_nominal_value=1  i_nominal_unit=A  v_specify=off  v_priority=None  v=0 V  v_nominal_specify=off  v_nominal_value=1  v_nominal_unit=V  vc_specify=on  vc_priority=High  vc=48 V  vc_nominal_specify=off  vc_nominal_value=1  vc_nominal_unit=V  T_specify=off  T_priority=None  T=298.15 K  T_nominal_specify=off  T_nominal_value=1  T_nominal_unit=K
      settings: AttributesFormatString=8x UR080M102J35TC97S00A: 8000uF, equivalent ESR 3.875mOhm
  COUT_HF_MLCC_Cap : ee_lib/Passive/Capacitor  cap_option=ee.enum.passive.capacitor.capOption.const  c=40 uF  Cvec=[1e-05, 1e-06] F  Vvec=[0, 10] V  CV_table_symmetry=ee.enum.passive.capacitor.tableSymmetry.yes  f_vec=[1, 10] kHz  DFext_vec=[.8, 1.2]  enable_C_tol=ee.enum.toleranceApplication.none  averaging_period=0 s  C_tol=5  tol_distribution=ee.enum.toleranceDistribution.uniform  nSigma=4  r=0.0005 Ohm  g=0 1/Ohm  enable_operating_limits=ee.enum.enable.no  operating_limit_action=ee.enum.passive.reportOpLim.warn  max_working_voltage_range=[-25, 25] V  power_rating=1 W  maxTemperature=85 degC  thermalEnable=false  thermalMass=1 J/K  fault_action=simscape.enum.assert.action.none  t_fault=1 s  i_specify=off  i_priority=None  i=0 A  i_nominal_specify=off  i_nominal_value=1  i_nominal_unit=A  v_specify=off  v_priority=None  v=0 V  v_nominal_specify=off  v_nominal_value=1  v_nominal_unit=V  vc_specify=on  vc_priority=High  vc=48 V  vc_nominal_specify=off  vc_nominal_value=1  vc_nominal_unit=V  T_specify=off  T_priority=None  T=298.15 K  T_nominal_specify=off  T_nominal_value=1  T_nominal_unit=K
      settings: AttributesFormatString=8x TDK C5750X7S2A106K230KE after LOUT; conservative 40uF effective total at 48V
  COUT_Y_Neg_to_PE : ee_lib/Passive/Capacitor  cap_option=ee.enum.passive.capacitor.capOption.const  c=2.2 nF  Cvec=[1e-05, 1e-06] F  Vvec=[0, 10] V  CV_table_symmetry=ee.enum.passive.capacitor.tableSymmetry.yes  f_vec=[1, 10] kHz  DFext_vec=[.8, 1.2]  enable_C_tol=ee.enum.toleranceApplication.none  averaging_period=0 s  C_tol=5  tol_distribution=ee.enum.toleranceDistribution.uniform  nSigma=4  r=0.02 Ohm  g=0 1/Ohm  enable_operating_limits=ee.enum.enable.no  operating_limit_action=ee.enum.passive.reportOpLim.warn  max_working_voltage_range=[-25, 25] V  power_rating=1 W  maxTemperature=85 degC  thermalEnable=false  thermalMass=1 J/K  fault_action=simscape.enum.assert.action.none  t_fault=1 s  i_specify=off  i_priority=None  i=0 A  i_nominal_specify=off  i_nominal_value=1  i_nominal_unit=A  v_specify=off  v_priority=None  v=0 V  v_nominal_specify=off  v_nominal_value=1  v_nominal_unit=V  vc_specify=off  vc_priority=High  vc=0 V  vc_nominal_specify=off  vc_nominal_value=1  vc_nominal_unit=V  T_specify=off  T_priority=None  T=298.15 K  T_nominal_specify=off  T_nominal_value=1  T_nominal_unit=K
      settings: AttributesFormatString=Y 2.2nF
  COUT_Y_Pos_to_PE : ee_lib/Passive/Capacitor  cap_option=ee.enum.passive.capacitor.capOption.const  c=2.2 nF  Cvec=[1e-05, 1e-06] F  Vvec=[0, 10] V  CV_table_symmetry=ee.enum.passive.capacitor.tableSymmetry.yes  f_vec=[1, 10] kHz  DFext_vec=[.8, 1.2]  enable_C_tol=ee.enum.toleranceApplication.none  averaging_period=0 s  C_tol=5  tol_distribution=ee.enum.toleranceDistribution.uniform  nSigma=4  r=0.02 Ohm  g=0 1/Ohm  enable_operating_limits=ee.enum.enable.no  operating_limit_action=ee.enum.passive.reportOpLim.warn  max_working_voltage_range=[-25, 25] V  power_rating=1 W  maxTemperature=85 degC  thermalEnable=false  thermalMass=1 J/K  fault_action=simscape.enum.assert.action.none  t_fault=1 s  i_specify=off  i_priority=None  i=0 A  i_nominal_specify=off  i_nominal_value=1  i_nominal_unit=A  v_specify=off  v_priority=None  v=0 V  v_nominal_specify=off  v_nominal_value=1  v_nominal_unit=V  vc_specify=off  vc_priority=High  vc=0 V  vc_nominal_specify=off  vc_nominal_value=1  vc_nominal_unit=V  T_specify=off  T_priority=None  T=298.15 K  T_nominal_specify=off  T_nominal_value=1  T_nominal_unit=K
      settings: AttributesFormatString=Y 2.2nF
  CSEC_DC_Link_Cap : ee_lib/Passive/Capacitor  cap_option=ee.enum.passive.capacitor.capOption.const  c=94 uF  Cvec=[1e-05, 1e-06] F  Vvec=[0, 10] V  CV_table_symmetry=ee.enum.passive.capacitor.tableSymmetry.yes  f_vec=[1, 10] kHz  DFext_vec=[.8, 1.2]  enable_C_tol=ee.enum.toleranceApplication.none  averaging_period=0 s  C_tol=5  tol_distribution=ee.enum.toleranceDistribution.uniform  nSigma=4  r=0.056 Ohm  g=0 1/Ohm  enable_operating_limits=ee.enum.enable.no  operating_limit_action=ee.enum.passive.reportOpLim.warn  max_working_voltage_range=[-100,100] V  power_rating=1 W  maxTemperature=85 degC  thermalEnable=false  thermalMass=1 J/K  fault_action=simscape.enum.assert.action.none  t_fault=1 s  i_specify=off  i_priority=None  i=0 A  i_nominal_specify=off  i_nominal_value=1  i_nominal_unit=A  v_specify=off  v_priority=None  v=0 V  v_nominal_specify=off  v_nominal_value=1  v_nominal_unit=V  vc_specify=on  vc_priority=High  vc=48 V  vc_nominal_specify=off  vc_nominal_value=1  vc_nominal_unit=V  T_specify=off  T_priority=None  T=298.15 K  T_nominal_specify=off  T_nominal_value=1  T_nominal_unit=K
      settings: AttributesFormatString=2x Panasonic EEUFS2A470 before LOUT: 94uF total, 56mOhm equivalent max impedance
  CSEC_HF_MLCC_Bank : ee_lib/Passive/Capacitor  cap_option=ee.enum.passive.capacitor.capOption.const  c=40 uF  Cvec=[1e-05, 1e-06] F  Vvec=[0, 10] V  CV_table_symmetry=ee.enum.passive.capacitor.tableSymmetry.yes  f_vec=[1, 10] kHz  DFext_vec=[.8, 1.2]  enable_C_tol=ee.enum.toleranceApplication.none  averaging_period=0 s  C_tol=5  tol_distribution=ee.enum.toleranceDistribution.uniform  nSigma=4  r=0.001 Ohm  g=0 1/Ohm  enable_operating_limits=ee.enum.enable.no  operating_limit_action=ee.enum.passive.reportOpLim.warn  max_working_voltage_range=[-25, 25] V  power_rating=1 W  maxTemperature=85 degC  thermalEnable=false  thermalMass=1 J/K  fault_action=simscape.enum.assert.action.none  t_fault=1 s  i_specify=off  i_priority=None  i=0 A  i_nominal_specify=off  i_nominal_value=1  i_nominal_unit=A  v_specify=off  v_priority=None  v=0 V  v_nominal_specify=off  v_nominal_value=1  v_nominal_unit=V  vc_specify=on  vc_priority=High  vc=48 V  vc_nominal_specify=off  vc_nominal_value=1  vc_nominal_unit=V  T_specify=off  T_priority=None  T=298.15 K  T_nominal_specify=off  T_nominal_value=1  T_nominal_unit=K
      settings: AttributesFormatString=8x TDK C5750X7S2A106K230KE before LOUT; conservative 40uF effective total at 48V
  Iout_To_Simulink : nesl_utility/PS-Simulink Converter  PhysicalDomain=network_engine_domain  SubClassName=ps_output  LeftPortType=input  RightPortType=output  PseudoPeriodic=off  Frequencies=[]  VectorFormat=inherit  Unit=inherit  AffineConversion=off
  Output_Current_Sensor : fl_lib/Electrical/Electrical Sensors/Current Sensor
      settings: AttributesFormatString=Iout sense
  ROUT_ACS725_1p2mOhm : ee_lib/Passive/Resistor  Description=ACS725 output-current sensor conductor resistance, not a shunt BOM part.  R=0.0012 Ohm  enable_R_tol=ee.enum.toleranceApplication.none  R_tol=5  tol_distribution=ee.enum.toleranceDistribution.uniform  nSigma=4  enable_operating_limits=ee.enum.enable.no  operating_limit_action=ee.enum.passive.reportOpLim.warn  power_rating=1 W  max_working_voltage=100 V  noise_mode=ee.enum.sources.noise.Disabled  Tdevice=25 degC  sample_time=1e-3 s  repeatability=ee.enum.ic.repeatability.notRepeatable  user_seed=0  auto_seed=3499211588  fault_action=simscape.enum.assert.action.none  t_fault=1 s  power_derating_T1=70 degC  power_derating_T2=155 degC  operating_temperature_range_vec=[-50, 150] degC  alpha=3.93e-3 1/K  Tmeas=25 degC  thermal_mass=100 J/K  temperature_specify=off  temperature_priority=High  temperature=298.15 K  temperature_nominal_specify=off  temperature_nominal_value=1  temperature_nominal_unit=K
      settings: AttributesFormatString=1mR
  ROUT_Bleeder : ee_lib/Passive/Resistor  R=4800 Ohm  enable_R_tol=ee.enum.toleranceApplication.none  R_tol=5  tol_distribution=ee.enum.toleranceDistribution.uniform  nSigma=4  enable_operating_limits=ee.enum.enable.no  operating_limit_action=ee.enum.passive.reportOpLim.warn  power_rating=1 W  max_working_voltage=100 V  noise_mode=ee.enum.sources.noise.Disabled  Tdevice=25 degC  sample_time=1e-3 s  repeatability=ee.enum.ic.repeatability.notRepeatable  user_seed=0  auto_seed=3298293894  fault_action=simscape.enum.assert.action.none  t_fault=1 s  power_derating_T1=70 degC  power_derating_T2=155 degC  operating_temperature_range_vec=[-50, 150] degC  alpha=3.93e-3 1/K  Tmeas=25 degC  thermal_mass=100 J/K  temperature_specify=off  temperature_priority=High  temperature=298.15 K  temperature_nominal_specify=off  temperature_nominal_value=1  temperature_nominal_unit=K
      settings: AttributesFormatString=2x 2.49kOhm 1W in series: 4.98kOhm output safety bleeder
  RPE_Output_Bleed : ee_lib/Passive/Resistor  R=100000000 Ohm  enable_R_tol=ee.enum.toleranceApplication.none  R_tol=5  tol_distribution=ee.enum.toleranceDistribution.uniform  nSigma=4  enable_operating_limits=ee.enum.enable.no  operating_limit_action=ee.enum.passive.reportOpLim.warn  power_rating=1 W  max_working_voltage=100 V  noise_mode=ee.enum.sources.noise.Disabled  Tdevice=25 degC  sample_time=1e-3 s  repeatability=ee.enum.ic.repeatability.notRepeatable  user_seed=0  auto_seed=2843506394  fault_action=simscape.enum.assert.action.none  t_fault=1 s  power_derating_T1=70 degC  power_derating_T2=155 degC  operating_temperature_range_vec=[-50, 150] degC  alpha=3.93e-3 1/K  Tmeas=25 degC  thermal_mass=100 J/K  temperature_specify=off  temperature_priority=High  temperature=298.15 K  temperature_nominal_specify=off  temperature_nominal_value=1  temperature_nominal_unit=K
      settings: AttributesFormatString=100MR
  Rload_DC_Output : ee_lib/Passive/Resistor  R=7.68 Ohm  enable_R_tol=ee.enum.toleranceApplication.none  R_tol=5  tol_distribution=ee.enum.toleranceDistribution.uniform  nSigma=4  enable_operating_limits=ee.enum.enable.no  operating_limit_action=ee.enum.passive.reportOpLim.warn  power_rating=1 W  max_working_voltage=100 V  noise_mode=ee.enum.sources.noise.Disabled  Tdevice=25 degC  sample_time=1e-3 s  repeatability=ee.enum.ic.repeatability.notRepeatable  user_seed=0  auto_seed=3320430498  fault_action=simscape.enum.assert.action.none  t_fault=1 s  power_derating_T1=70 degC  power_derating_T2=155 degC  operating_temperature_range_vec=[-50, 150] degC  alpha=3.93e-3 1/K  Tmeas=25 degC  thermal_mass=100 J/K  temperature_specify=off  temperature_priority=High  temperature=298.15 K  temperature_nominal_specify=off  temperature_nominal_value=1  temperature_nominal_unit=K
      settings: AttributesFormatString=Rload
  SEC_Return_Ref : fl_lib/Electrical/Electrical Elements/Electrical Reference
  Vout_Sensor : fl_lib/Electrical/Electrical Sensors/Voltage Sensor
      settings: AttributesFormatString=Vout sense
  Vout_To_Simulink : nesl_utility/PS-Simulink Converter  PhysicalDomain=network_engine_domain  SubClassName=ps_output  LeftPortType=input  RightPortType=output  PseudoPeriodic=off  Frequencies=[]  VectorFormat=inherit  Unit=inherit  AffineConversion=off
  Conn1 : PMIOPort  Side=Right
  Conn2 : PMIOPort  Port=2  Side=Right
  output : Outport
  output1 : Outport  Port=2
  wires:
  Vout_To_Simulink/1 -> output/1
  Iout_To_Simulink/1 -> output1/1
  connections:
  CSEC_DC_Link_Cap/RConn1 -- CSEC_HF_MLCC_Bank/RConn1 -- ROUT_Bleeder/RConn1 -- Vout_Sensor/RConn2 -- Rload_DC_Output/RConn1 -- COUT_HF_MLCC_Cap/RConn1 -- COUT_Y_Neg_to_PE/LConn1 -- Conn2/RConn1 -- RPE_Output_Bleed/RConn1 -- SEC_Return_Ref/LConn1 -- COUT_DC_Bulk/RConn1
  Vout_Sensor/RConn1 -- Vout_To_Simulink/LConn1
  Output_Current_Sensor/RConn1 -- Iout_To_Simulink/LConn1
  COUT_Y_Pos_to_PE/RConn1 -- COUT_Y_Neg_to_PE/RConn1 -- RPE_Output_Bleed/LConn1
  Output_Current_Sensor/LConn1 -- COUT_DC_Bulk/LConn1 -- CSEC_DC_Link_Cap/LConn1 -- CSEC_HF_MLCC_Bank/LConn1 -- Conn1/RConn1
  Output_Current_Sensor/RConn2 -- ROUT_ACS725_1p2mOhm/LConn1
  Vout_Sensor/LConn1 -- ROUT_ACS725_1p2mOhm/RConn1 -- ROUT_Bleeder/LConn1 -- COUT_Y_Pos_to_PE/LConn1 -- COUT_HF_MLCC_Cap/LConn1 -- Rload_DC_Output/LConn1

== system DAB_RA8P1_Final_Physical_MOSFET/PRI_Full_Bridge_RealDrivers ==
  note: Left: DC bus and isolated gate inputs. Right: switch nodes to transformer. Each leg contains two real FET blocks.
  G1_A_HS : Inport
  G2_A_LS : Inport  Port=2
  G3_B_HS : Inport  Port=3
  G4_B_LS : Inport  Port=4
  Leg_A_RealSwitchingCell : Subsystem
      mask Display: color('black');disp('Leg A RealSwitchingCell\nHS/LS nonideal FETs');
  Leg_B_RealSwitchingCell : Subsystem
      mask Display: color('black');disp('Leg B RealSwitchingCell\nHS/LS nonideal FETs');
  P_BUS : PMIOPort  Side=Left
  N_BUS : PMIOPort  Port=2  Side=Left
  SW_A : PMIOPort  Port=3  Side=Right
  SW_B : PMIOPort  Port=4  Side=Right
  wires:
  G1_A_HS/1 -> Leg_A_RealSwitchingCell/1(G_HS)
  G2_A_LS/1 -> Leg_A_RealSwitchingCell/2(G_LS)
  G3_B_HS/1 -> Leg_B_RealSwitchingCell/1(G_HS)
  G4_B_LS/1 -> Leg_B_RealSwitchingCell/2(G_LS)
  connections:
  Leg_A_RealSwitchingCell/LConn1 -- P_BUS/RConn1 -- Leg_B_RealSwitchingCell/LConn1
  Leg_A_RealSwitchingCell/LConn2 -- N_BUS/RConn1 -- Leg_B_RealSwitchingCell/LConn2
  Leg_A_RealSwitchingCell/RConn1 -- SW_A/RConn1
  Leg_B_RealSwitchingCell/RConn1 -- SW_B/RConn1
